simulink model "scheme_L2"  (R2025b)
settings: Solver=VariableStepAuto  StartTime=0.0  StopTime=10.0  RelTol=1e-3
settings Model: Creator=markg  LastModifiedBy=markg

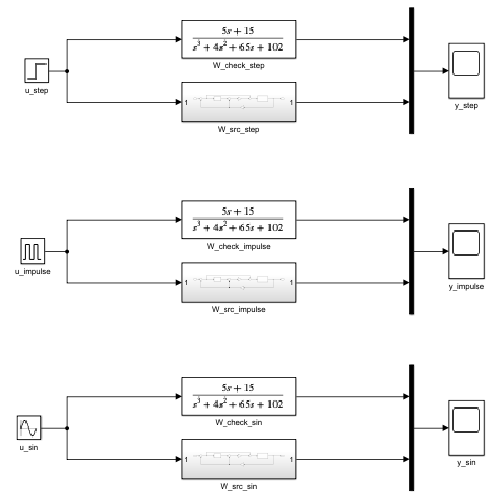
[thumbnail: Simulink's stored preview of the top-level diagram]
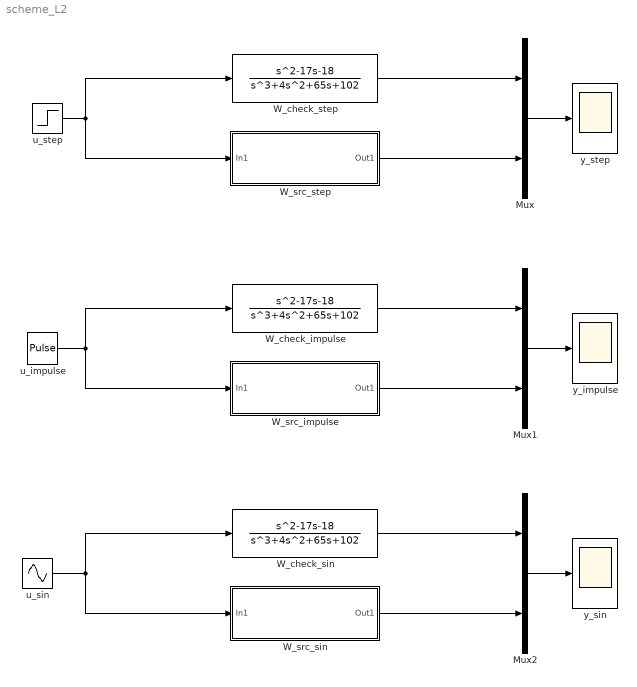
== system scheme_L2 ==
  Mux : Mux  Inputs=2
  Mux1 : Mux  Inputs=2
  Mux2 : Mux  Inputs=2
  W_check_impulse : TransferFcn  Numerator=[1 -17 -18]  Denominator=[1 4 65 102]
  W_check_sin : TransferFcn  Numerator=[1 -17 -18]  Denominator=[1 4 65 102]
  W_check_step : TransferFcn  Numerator=[1 -17 -18]  Denominator=[1 4 65 102]
  W_src_impulse : Subsystem
  W_src_sin : Subsystem
  W_src_step : Subsystem
  u_impulse : DiscretePulseGenerator  PulseType=Time based  Period=10  PulseWidth=5  PhaseDelay=1
  u_sin : Sin  Frequency=2  SampleTime=0
  u_step : Step  SampleTime=0
  y_impulse : Scope
      settings: ActiveDisplayYMinimum=-0.6  ActiveDisplayYMaximum=0.5
  y_sin : Scope
      settings: ActiveDisplayYMinimum=-0.6  ActiveDisplayYMaximum=0.5  DataLoggingVariableName=ScopeData2
  y_step : Scope
      settings: ActiveDisplayYMinimum=-0.6  ActiveDisplayYMaximum=0.5
  wires:
  u_step/1 -> W_src_step/1(In1), W_check_step/1
  Mux/1 -> y_step/1
  W_src_step/1(Out1) -> Mux/2
  W_check_step/1 -> Mux/1
  W_src_impulse/1(Out1) -> Mux1/2
  u_impulse/1 -> W_src_impulse/1(In1), W_check_impulse/1
  Mux1/1 -> y_impulse/1
  W_check_impulse/1 -> Mux1/1
  W_src_sin/1(Out1) -> Mux2/2
  u_sin/1 -> W_src_sin/1(In1), W_check_sin/1
  W_check_sin/1 -> Mux2/1
  Mux2/1 -> y_sin/1

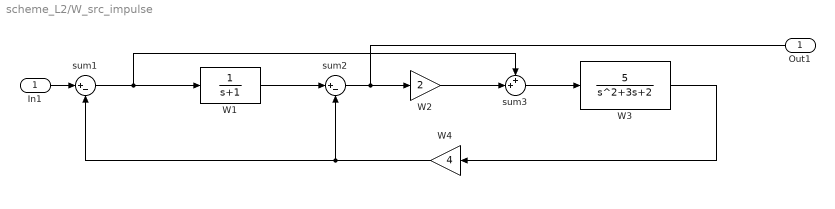
== system scheme_L2/W_src_impulse ==
  In1 : Inport
  W1 : TransferFcn  Denominator=[1 1]
  W2 : Gain  Gain=2
  W3 : TransferFcn  Numerator=[5]  Denominator=[1 3 2]
  W4 : Gain  Gain=4
  sum1 : Sum  Inputs=|+-
  sum2 : Sum  Inputs=|+-
  sum3 : Sum  Inputs=++|
  Out1 : Outport
  wires:
  W1/1 -> sum2/1
  W3/1 -> W4/1
  W4/1 -> sum1/2, sum2/2
  sum1/1 -> sum3/1, W1/1
  sum2/1 -> W2/1, Out1/1
  sum3/1 -> W3/1
  In1/1 -> sum1/1
  W2/1 -> sum3/2

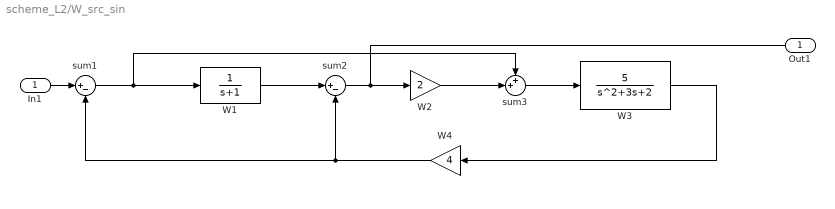
== system scheme_L2/W_src_sin ==
  In1 : Inport
  W1 : TransferFcn  Denominator=[1 1]
  W2 : Gain  Gain=2
  W3 : TransferFcn  Numerator=[5]  Denominator=[1 3 2]
  W4 : Gain  Gain=4
  sum1 : Sum  Inputs=|+-
  sum2 : Sum  Inputs=|+-
  sum3 : Sum  Inputs=++|
  Out1 : Outport
  wires:
  W1/1 -> sum2/1
  W3/1 -> W4/1
  W4/1 -> sum1/2, sum2/2
  sum1/1 -> sum3/1, W1/1
  sum2/1 -> W2/1, Out1/1
  sum3/1 -> W3/1
  In1/1 -> sum1/1
  W2/1 -> sum3/2

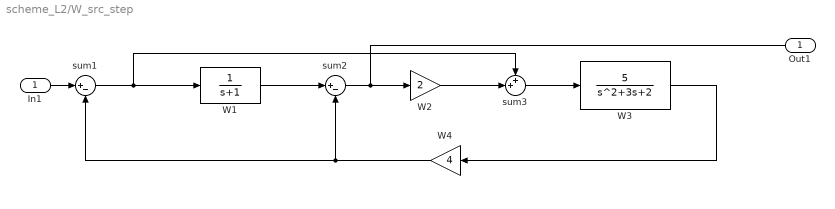
== system scheme_L2/W_src_step ==
  In1 : Inport
  W1 : TransferFcn  Denominator=[1 1]
  W2 : Gain  Gain=2
  W3 : TransferFcn  Numerator=[5]  Denominator=[1 3 2]
  W4 : Gain  Gain=4
  sum1 : Sum  Inputs=|+-
  sum2 : Sum  Inputs=|+-
  sum3 : Sum  Inputs=++|
  Out1 : Outport
  wires:
  W1/1 -> sum2/1
  W3/1 -> W4/1
  W4/1 -> sum1/2, sum2/2
  sum1/1 -> sum3/1, W1/1
  sum2/1 -> W2/1, Out1/1
  sum3/1 -> W3/1
  In1/1 -> sum1/1
  W2/1 -> sum3/2
